simulink model "L3_POLI_ZEROURI_Kp_schimbat"  (R2025b)
settings: Solver=VariableStepAuto  StartTime=0.0  StopTime=20  RelTol=1e-3
settings Model: Creator=anama  LastModifiedBy=elisa

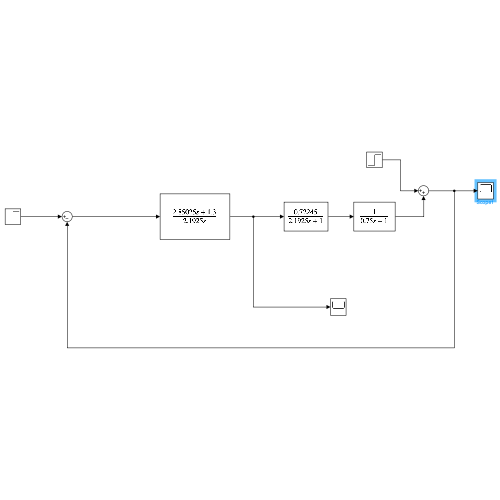
[thumbnail: Simulink's stored preview of the top-level diagram]
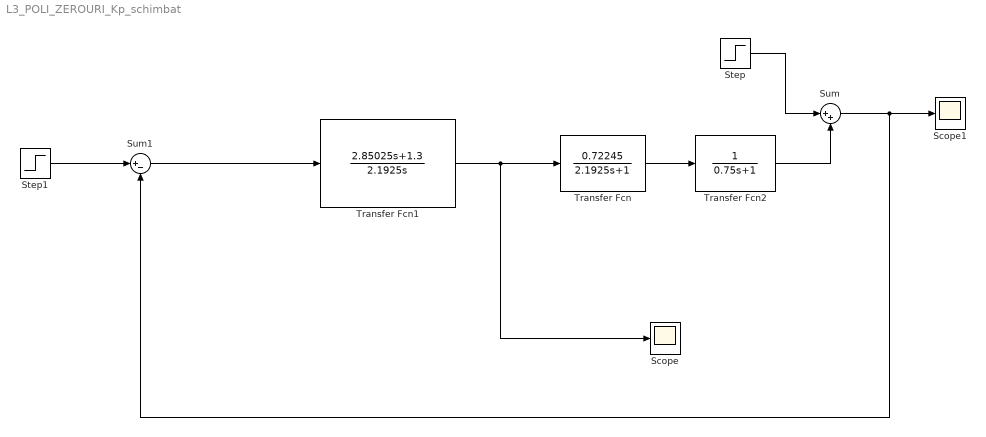
== system L3_POLI_ZEROURI_Kp_schimbat ==
  Scope : Scope
      settings: ActiveDisplayYMinimum=125.77332417342853  ActiveDisplayYMaximum=168.04008243914319
  Scope1 : Scope
      settings: ActiveDisplayYMinimum=-2.5347503059554377  ActiveDisplayYMaximum=122.81275275359897
  Step : Step  Time=0  After=10  SampleTime=0
  Step1 : Step  Time=0  After=110  SampleTime=0
  Sum : Sum  Inputs=|++
  Sum1 : Sum  Inputs=|+-
  Transfer Fcn : TransferFcn  Numerator=[0.72245]  Denominator=[2.1925 1]
  Transfer Fcn1 : TransferFcn  Numerator=[2.85025 1.3]  Denominator=[2.1925 0]
  Transfer Fcn2 : TransferFcn  Denominator=[0.75 1]
  wires:
  Transfer Fcn/1 -> Transfer Fcn2/1
  Step/1 -> Sum/1
  Transfer Fcn2/1 -> Sum/2
  Sum/1 -> Sum1/2, Scope1/1
  Transfer Fcn1/1 -> Scope/1, Transfer Fcn/1
  Sum1/1 -> Transfer Fcn1/1
  Step1/1 -> Sum1/1
